simulink model "Template_v5_0_0_2026a_Original"  (R2026a)
settings: Solver=ode4  StopTime=tsim  FixedStep=baseRate  RelTol=1e-6  AbsTol=1e-6
undefined symbols (not defined in the file or in its folder): baseRate, dataRate, DiscIntNeverNeededParam, F_thrusters_BLACK, F_thrusters_BLUE, F_thrusters_RED, home_states_BLACK, home_states_BLUE, home_states_RED, IBLACK, IBLUE, init_states_BLACK, init_states_BLUE, init_states_RED, IRED, K_BLACK, K_BLUE, K_RED, labConsoleIP, mBLACK, mBLUE, mRED, Phase0_End, Phase1_End, Phase2_End, Phase3_End, Phase3_SubPhase1_End, Phase3_SubPhase2_End, Phase3_SubPhase3_End, Phase3_SubPhase4_End, Phase4_End, Phase5_End, platformSelection, PWMFreq, serverRate, simMode, tableDamping_BLACK, tableDamping_BLUE, tableDamping_RED, tableSlope, thrust_decay_BLACK, thrust_decay_BLUE, thrust_decay_RED, thruster_dist2CG_BLACK, thruster_dist2CG_BLUE, thruster_dist2CG_RED, xLength, yLength
libraries: simulink x18, dspinverses x3, nvidiaCommlib x1
(part 5 of 7)

== system Template_v5_0_0_2026a_Original/Simulate Plant Dynamics/BLUE Dynamics/Calculated & Store Measured States/Subsystem1 ==
  dt : Inport
  y : Inport  Port=2
  Constant3 : Constant  Value=0
  Delay1 : Delay  DelayLength=1
  Enabled Subsystem : Subsystem  TreatAsAtomicUnit=on
  Relational Operator : RelationalOperator  Operator=~=  OutDataTypeStr=boolean  RndMeth=Simplest  InputSameDT=off
  Subtract1 : Sum  Inputs=+-
  dy/dt : Outport
  wires:
  Constant3/1 -> Relational Operator/2
  Relational Operator/1 -> Enabled Subsystem/Enable
  Delay1/1 -> Subtract1/2
  dt/1 -> Enabled Subsystem/2(dt)
  Subtract1/1 -> Relational Operator/1
  Enabled Subsystem/1(dy/dt) -> dy/dt/1
  y/1 -> Enabled Subsystem/1(y), Delay1/1, Subtract1/1

== system Template_v5_0_0_2026a_Original/Simulate Plant Dynamics/BLUE Dynamics/Calculated & Store Measured States/Subsystem2 ==
  dt : Inport
  y : Inport  Port=2
  Constant3 : Constant  Value=0
  Delay1 : Delay  DelayLength=1
  Enabled Subsystem : Subsystem  TreatAsAtomicUnit=on
  Relational Operator : RelationalOperator  Operator=~=  OutDataTypeStr=boolean  RndMeth=Simplest  InputSameDT=off
  Subtract1 : Sum  Inputs=+-
  dy/dt : Outport
  wires:
  Constant3/1 -> Relational Operator/2
  Relational Operator/1 -> Enabled Subsystem/Enable
  Delay1/1 -> Subtract1/2
  dt/1 -> Enabled Subsystem/2(dt)
  Subtract1/1 -> Relational Operator/1
  Enabled Subsystem/1(dy/dt) -> dy/dt/1
  y/1 -> Enabled Subsystem/1(y), Delay1/1, Subtract1/1

== system Template_v5_0_0_2026a_Original/Simulate Plant Dynamics/BLUE Dynamics/Calculated & Store Measured States/Wrap ==
  Unwrapped Angle : Inport
  Atan2 : Trigonometry  Operator=atan2
  Cos : Trigonometry  Operator=cos
  Sin : Trigonometry
  Wrapped Angle : Outport
  wires:
  Unwrapped Angle/1 -> Sin/1, Cos/1
  Cos/1 -> Atan2/2
  Atan2/1 -> Wrapped Angle/1
  Sin/1 -> Atan2/1

== system Template_v5_0_0_2026a_Original/Simulate Plant Dynamics/BLUE Dynamics/Calculated & Store True States/Wrap ==
  Unwrapped Angle : Inport
  Atan2 : Trigonometry  Operator=atan2
  Cos : Trigonometry  Operator=cos
  Sin : Trigonometry
  Wrapped Angle : Outport
  wires:
  Unwrapped Angle/1 -> Sin/1, Cos/1
  Cos/1 -> Atan2/2
  Atan2/1 -> Wrapped Angle/1
  Sin/1 -> Atan2/1

== system Template_v5_0_0_2026a_Original/Simulate Plant Dynamics/BLUE Dynamics/Data @ Measurement Rate/Calculate True Time Step ==
  Data : Inport
  Time : Inport  Port=2
  Rate : Inport  Port=3
  Constant3 : Constant  Value=0
  Delay1 : Delay  DelayLength=1  InitialCondition=0
  Delay2 : Delay  DelayLength=1  InitialCondition=0
  Demux : Demux  Outputs=3
  Enabled Subsystem3 : Subsystem  TreatAsAtomicUnit=on
  MATLAB Function : MATLAB Function  TreatAsAtomicUnit=on
  Relational Operator : RelationalOperator  Operator=~=  OutDataTypeStr=boolean  RndMeth=Simplest  InputSameDT=off
  Subtract1 : Sum  Inputs=+-
  Subtract2 : Sum  Inputs=+-
  Terminator : Terminator
  Terminator1 : Terminator
  dt_out : Outport
  wires:
  Demux/3 -> Terminator1/1
  Rate/1 -> MATLAB Function/2(dataRate)
  MATLAB Function/1(dt_out) -> dt_out/1
  Time/1 -> Delay2/1, Subtract1/1
  Enabled Subsystem3/1(dy(t)/dt) -> MATLAB Function/1(dt)
  Data/1 -> Demux/1
  Subtract2/1 -> Relational Operator/1
  Relational Operator/1 -> Enabled Subsystem3/Enable
  Constant3/1 -> Relational Operator/2
  Demux/1 -> Subtract2/1, Delay1/1
  Delay1/1 -> Subtract2/2
  Demux/2 -> Terminator/1
  Subtract1/1 -> Enabled Subsystem3/1(y2-y1)
  Delay2/1 -> Subtract1/2

== system Template_v5_0_0_2026a_Original/Simulate Plant Dynamics/BLUE Dynamics/Data @ Measurement Rate/Enabled Subsystem ==
  In1 : Inport
  Enable : EnablePort
  Out1 : Outport
  wires:
  In1/1 -> Out1/1

== system Template_v5_0_0_2026a_Original/Simulate Plant Dynamics/BLUE Dynamics/Data @ Measurement Rate/Enabled Subsystem1 ==
  ThrustPer_Final : Inport
  Enable : EnablePort
  Out1 : Outport
  wires:
  ThrustPer_Final/1 -> Out1/1

== system Template_v5_0_0_2026a_Original/Simulate Plant Dynamics/RED and ARM Dynamics/RED + ARM/Calculated & Store Measured States ==
  y : Inport
  dt : Inport  Port=2
  Arm (Stored by the Encoder Path) : Terminator
  Demux1 : Demux  Outputs=3
  Demux2 : Demux  Outputs=[3,3]
  Mux3 : Mux  Inputs=3
  Mux4 : Mux  Inputs=3
  Mux5 : Mux  Inputs=2
  Reshape1 : Reshape  OutputDimensionality=Column vector (2-D)
  Subsystem3 : Subsystem
  Subsystem4 : Subsystem
  Subsystem5 : Subsystem
  True States for RED : DataStoreWrite  DataStoreName=RED_Measured_States  IndexOptions=Index vector (dialog)  Indices=1  OutputSizes=1
  Wrap : Subsystem
  wires:
  Demux1/2 -> Mux3/2
  Wrap/1(Wrapped Angle) -> Mux3/3
  Demux2/1 -> Subsystem3/2(y), Demux1/1
  Mux4/1 -> True States for RED/1
  y/1 -> Demux2/1
  Subsystem5/1(dy/dt) -> Mux5/2
  Demux1/1 -> Mux3/1
  Demux2/2 -> Subsystem5/2(y), Mux5/1
  Mux3/1 -> Mux4/1
  Subsystem4/1(dy/dt) -> Mux4/3
  Demux1/3 -> Wrap/1(Unwrapped Angle)
  dt/1 -> Subsystem5/1(dt), Subsystem4/1(dt), Subsystem3/1(dt)
  Reshape1/1 -> Subsystem4/2(y)
  Subsystem3/1(dy/dt) -> Mux4/2, Reshape1/1
  Mux5/1 -> Arm (Stored by the Encoder Path)/1

== system Template_v5_0_0_2026a_Original/Simulate Plant Dynamics/RED and ARM Dynamics/RED + ARM/Calculated & Store True States ==
  y : Inport
  Data Store Write3 : DataStoreWrite  DataStoreName=ARM_True_States  IndexOptions=Index vector (dialog)  Indices=1  OutputSizes=1
  Demux : Demux  Outputs=3
  Demux1 : Demux  Outputs=[3,3]
  Discrete Derivative : simulink/Discrete/Discrete Derivative  gainval=1.0  ICPrevScaledInput=0.0  OutMin=[]  OutMax=[]  OutDataType=fixdt(1, 16)  OutScaling=2^-10  DoSatur=off
  Discrete Derivative1 : simulink/Discrete/Discrete Derivative  gainval=1.0  ICPrevScaledInput=0.0  OutMin=[]  OutMax=[]  OutDataType=fixdt(1, 16)  OutScaling=2^-10  DoSatur=off
  Discrete Derivative2 : simulink/Discrete/Discrete Derivative  gainval=1.0  ICPrevScaledInput=0.0  OutMin=[]  OutMax=[]  OutDataType=fixdt(1, 16)  OutScaling=2^-10  DoSatur=off
  Mux1 : Mux  Inputs=3
  Mux2 : Mux  Inputs=3
  Mux3 : Mux  Inputs=2
  True States for RED : DataStoreWrite  DataStoreName=RED_True_States  IndexOptions=Index vector (dialog)  Indices=1  OutputSizes=1
  Wrap : Subsystem
  wires:
  Demux/1 -> Mux1/1
  Wrap/1(Wrapped Angle) -> Mux1/3
  Demux/3 -> Wrap/1(Unwrapped Angle)
  Demux/2 -> Mux1/2
  Mux2/1 -> True States for RED/1
  Discrete Derivative/1 -> Discrete Derivative1/1, Mux2/2
  Mux1/1 -> Mux2/1
  Discrete Derivative1/1 -> Mux2/3
  y/1 -> Demux1/1
  Demux1/1 -> Discrete Derivative/1, Demux/1
  Mux3/1 -> Data Store Write3/1
  Demux1/2 -> Discrete Derivative2/1, Mux3/1
  Discrete Derivative2/1 -> Mux3/2

== system Template_v5_0_0_2026a_Original/Simulate Plant Dynamics/RED and ARM Dynamics/RED + ARM/Data @ Measurement Rate ==
  Data Input : Inport
  Calculate True Time Step : Subsystem
  Constant1 : Constant  Value=dataRate
  Constant2 : Constant  Value=0
  Data Store Read : DataStoreRead  DataStoreName=Univ_Time  IndexOptions=Index vector (dialog)  Indices=1  OutputSizes=1
  Delay : Delay  DelayLength=1
  Enabled Subsystem : Subsystem  TreatAsAtomicUnit=on
  Enabled Subsystem1 : Subsystem  TreatAsAtomicUnit=on
  Relational Operator1 : RelationalOperator  OutDataTypeStr=boolean  RndMeth=Simplest  InputSameDT=off
  Relational Operator2 : RelationalOperator  Operator===  OutDataTypeStr=boolean  RndMeth=Simplest  InputSameDT=off
  Subtract : Sum  Inputs=+-
  Data Held : Outport
  Time Step : Outport  Port=2
  wires:
  Data Input/1 -> Enabled Subsystem1/1(ThrustPer_Final)
  Subtract/1 -> Relational Operator2/1, Delay/1
  Relational Operator2/1 -> Enabled Subsystem1/Enable
  Relational Operator1/1 -> Enabled Subsystem/Enable
  Constant1/1 -> Calculate True Time Step/3(Rate), Relational Operator1/2
  Constant2/1 -> Relational Operator2/2
  Enabled Subsystem/1(Out1) -> Calculate True Time Step/2(Time), Subtract/2
  Delay/1 -> Relational Operator1/1
  Data Store Read/1 -> Enabled Subsystem/1(In1), Subtract/1
  Enabled Subsystem1/1(Out1) -> Calculate True Time Step/1(Data), Data Held/1
  Calculate True Time Step/1(dt_out) -> Time Step/1

== system Template_v5_0_0_2026a_Original/Simulate Plant Dynamics/RED and ARM Dynamics/RED + ARM/Exceeded Table Limits ==
  X : Inport
  Y : Inport  Port=2
  Constant : Constant  Value=xLength
  Constant1 : Constant  Value=0
  Constant2 : Constant  Value=yLength
  Constant3 : Constant  Value=0
  Logical Operator : Logic  Operator=OR  AllPortsSameDT=off  OutDataTypeStr=boolean
  Logical Operator1 : Logic  Operator=OR  AllPortsSameDT=off  OutDataTypeStr=boolean
  Logical Operator2 : Logic  Operator=OR  AllPortsSameDT=off  OutDataTypeStr=boolean
  Relational Operator : RelationalOperator  OutDataTypeStr=boolean  RndMeth=Simplest  InputSameDT=off
  Relational Operator1 : RelationalOperator  Operator=<  OutDataTypeStr=boolean  RndMeth=Simplest  InputSameDT=off
  Relational Operator2 : RelationalOperator  OutDataTypeStr=boolean  RndMeth=Simplest  InputSameDT=off
  Relational Operator3 : RelationalOperator  Operator=<  OutDataTypeStr=boolean  RndMeth=Simplest  InputSameDT=off
  Stop : Outport
  wires:
  Constant1/1 -> Relational Operator1/2
  Relational Operator/1 -> Logical Operator/1
  Relational Operator1/1 -> Logical Operator/2
  Constant/1 -> Relational Operator/2
  X/1 -> Relational Operator1/1, Relational Operator/1
  Relational Operator3/1 -> Logical Operator1/2
  Relational Operator2/1 -> Logical Operator1/1
  Constant3/1 -> Relational Operator3/2
  Constant2/1 -> Relational Operator2/2
  Y/1 -> Relational Operator3/1, Relational Operator2/1
  Logical Operator2/1 -> Stop/1
  Logical Operator/1 -> Logical Operator2/1
  Logical Operator1/1 -> Logical Operator2/2

== system Template_v5_0_0_2026a_Original/Simulate Plant Dynamics/RED and ARM Dynamics/RED Only/Calculated & Store Measured States ==
  y : Inport
  dt : Inport  Port=2
  Demux : Demux  Outputs=3
  Measured States for RED : DataStoreWrite  DataStoreName=RED_Measured_States  IndexOptions=Index vector (dialog)  Indices=1  OutputSizes=1
  Mux1 : Mux  Inputs=3
  Mux2 : Mux  Inputs=3
  Reshape : Reshape  OutputDimensionality=Column vector (2-D)
  Subsystem1 : Subsystem
  Subsystem2 : Subsystem
  Wrap : Subsystem
  wires:
  Demux/1 -> Mux1/1
  Wrap/1(Wrapped Angle) -> Mux1/3
  Demux/3 -> Wrap/1(Unwrapped Angle)
  Demux/2 -> Mux1/2
  Reshape/1 -> Subsystem1/2(y)
  dt/1 -> Subsystem2/1(dt), Subsystem1/1(dt)
  y/1 -> Subsystem2/2(y), Demux/1
  Mux1/1 -> Mux2/1
  Subsystem1/1(dy/dt) -> Mux2/3
  Mux2/1 -> Measured States for RED/1
  Subsystem2/1(dy/dt) -> Mux2/2, Reshape/1

== system Template_v5_0_0_2026a_Original/Simulate Plant Dynamics/RED and ARM Dynamics/RED Only/Calculated & Store True States ==
  y : Inport
  Demux : Demux  Outputs=3
  Discrete Derivative : simulink/Discrete/Discrete Derivative  gainval=1.0  ICPrevScaledInput=0.0  OutMin=[]  OutMax=[]  OutDataType=fixdt(1, 16)  OutScaling=2^-10  DoSatur=off
  Discrete Derivative1 : simulink/Discrete/Discrete Derivative  gainval=1.0  ICPrevScaledInput=0.0  OutMin=[]  OutMax=[]  OutDataType=fixdt(1, 16)  OutScaling=2^-10  DoSatur=off
  Mux1 : Mux  Inputs=3
  Mux2 : Mux  Inputs=3
  True States for RED : DataStoreWrite  DataStoreName=RED_True_States  IndexOptions=Index vector (dialog)  Indices=1  OutputSizes=1
  Wrap : Subsystem
  wires:
  Demux/1 -> Mux1/1
  Wrap/1(Wrapped Angle) -> Mux1/3
  Demux/3 -> Wrap/1(Unwrapped Angle)
  Demux/2 -> Mux1/2
  Mux2/1 -> True States for RED/1
  y/1 -> Discrete Derivative/1, Demux/1
  Discrete Derivative/1 -> Mux2/2, Discrete Derivative1/1
  Mux1/1 -> Mux2/1
  Discrete Derivative1/1 -> Mux2/3

== system Template_v5_0_0_2026a_Original/Simulate Plant Dynamics/RED and ARM Dynamics/RED Only/Data @ Measurement Rate ==
  Data Input : Inport
  Calculate True Time Step : Subsystem
  Constant1 : Constant  Value=dataRate
  Constant2 : Constant  Value=0
  Data Store Read : DataStoreRead  DataStoreName=Univ_Time  IndexOptions=Index vector (dialog)  Indices=1  OutputSizes=1
  Delay : Delay  DelayLength=1
  Enabled Subsystem : Subsystem  TreatAsAtomicUnit=on
  Enabled Subsystem1 : Subsystem  TreatAsAtomicUnit=on
  Relational Operator1 : RelationalOperator  OutDataTypeStr=boolean  RndMeth=Simplest  InputSameDT=off
  Relational Operator2 : RelationalOperator  Operator===  OutDataTypeStr=boolean  RndMeth=Simplest  InputSameDT=off
  Subtract : Sum  Inputs=+-
  Data Held : Outport
  Time Step : Outport  Port=2
  wires:
  Data Input/1 -> Enabled Subsystem1/1(ThrustPer_Final)
  Subtract/1 -> Relational Operator2/1, Delay/1
  Relational Operator2/1 -> Enabled Subsystem1/Enable
  Relational Operator1/1 -> Enabled Subsystem/Enable
  Constant1/1 -> Calculate True Time Step/3(Rate), Relational Operator1/2
  Constant2/1 -> Relational Operator2/2
  Enabled Subsystem/1(Out1) -> Calculate True Time Step/2(Time), Subtract/2
  Delay/1 -> Relational Operator1/1
  Data Store Read/1 -> Enabled Subsystem/1(In1), Subtract/1
  Enabled Subsystem1/1(Out1) -> Calculate True Time Step/1(Data), Data Held/1
  Calculate True Time Step/1(dt_out) -> Time Step/1

== system Template_v5_0_0_2026a_Original/Simulate Plant Dynamics/RED and ARM Dynamics/RED Only/Dynamics Model for RED ==
  control_inputs : Inport
  Acceleration to Velocity : DiscreteIntegrator  IntegratorMethod=Integration: Backward Euler  SampleTime=-1  ICPrevOutput=DiscIntNeverNeededParam  ICPrevScaledInput=DiscIntNeverNeededParam
  Float State : DataStoreRead  DataStoreName=Float_State  IndexOptions=Index vector (dialog)  Indices=1  OutputSizes=1
  MATLAB Function : MATLAB Function  TreatAsAtomicUnit=on
  Previous Position : UnitDelay  InitialCondition=init_states_RED(:)  SampleTime=-1
  Previous Velocity : UnitDelay  InitialCondition=[0; 0; 0]  SampleTime=-1
  Velocity to Position : DiscreteIntegrator  IntegratorMethod=Integration: Backward Euler  InitialCondition=init_states_RED  SampleTime=-1  ICPrevOutput=DiscIntNeverNeededParam  ICPrevScaledInput=DiscIntNeverNeededParam
  states : Outport  VectorParamsAs1DForOutWhenUnconnected=off
  wires:
  control_inputs/1 -> MATLAB Function/1(control_inputs)
  MATLAB Function/1(x_ddot) -> Acceleration to Velocity/1
  Acceleration to Velocity/1 -> Velocity to Position/1, Previous Velocity/1
  Velocity to Position/1 -> states/1, Previous Position/1
  Previous Position/1 -> MATLAB Function/2(position)
  Previous Velocity/1 -> MATLAB Function/3(velocity)
  Float State/1 -> MATLAB Function/4(floating)

== system Template_v5_0_0_2026a_Original/Thruster & Float Control Code/Change BLACK Behavior/Calculate Duty Cycle/Duty Cycle @ PWM ==
  ThrustPer_Final : Inport
  Constant1 : Constant  Value=1/PWMFreq
  Constant2 : Constant  Value=0
  Data Store Read : DataStoreRead  DataStoreName=Univ_Time  IndexOptions=Index vector (dialog)  Indices=1  OutputSizes=1
  Delay : Delay  DelayLength=1
  Enabled Subsystem : Subsystem  TreatAsAtomicUnit=on
  Enabled Subsystem1 : Subsystem  TreatAsAtomicUnit=on
  Relational Operator1 : RelationalOperator  OutDataTypeStr=boolean  RndMeth=Simplest  InputSameDT=off
  Relational Operator2 : RelationalOperator  Operator===  OutDataTypeStr=boolean  RndMeth=Simplest  InputSameDT=off
  Subtract : Sum  Inputs=+-
  Duty Cycle Held : Outport
  wires:
  Data Store Read/1 -> Enabled Subsystem/1(In1), Subtract/1
  ThrustPer_Final/1 -> Enabled Subsystem1/1(ThrustPer_Final)
  Subtract/1 -> Relational Operator2/1, Delay/1
  Relational Operator2/1 -> Enabled Subsystem1/Enable
  Relational Operator1/1 -> Enabled Subsystem/Enable
  Constant1/1 -> Relational Operator1/2
  Constant2/1 -> Relational Operator2/2
  Enabled Subsystem/1(Out1) -> Subtract/2
  Enabled Subsystem1/1(Out1) -> Duty Cycle Held/1
  Delay/1 -> Relational Operator1/1

== system Template_v5_0_0_2026a_Original/Thruster & Float Control Code/Change BLACK Behavior/Calculate Duty Cycle/Generate Initial Guess ==
  "[Fx; Fy; Tz]" : Inport
  MATLAB Function : MATLAB Function  TreatAsAtomicUnit=on
  Product3 : Product  Multiplication=Matrix(*)
  Pseudoinverse1 : dspinverses/Pseudoinverse  wanterr=off  SimulateUsing=Interpreted execution
  Duty Cycle : Outport
  wires:
  Pseudoinverse1/1 -> Product3/1
  MATLAB Function/1(H) -> Pseudoinverse1/1
  Product3/1 -> Duty Cycle/1
  "[Fx; Fy; Tz]"/1 -> Product3/2

== system Template_v5_0_0_2026a_Original/Thruster & Float Control Code/Change BLACK Behavior/Calculate Duty Cycle/Rotate Forces to Inertial ==
  "F_b " : Inport
  Rz : Inport  Port=2
  Create Rotation Matrix : MATLAB Function  TreatAsAtomicUnit=on
  Rotate F_b to F_I : Product  Multiplication=Matrix(*)
  F_I : Outport  VectorParamsAs1DForOutWhenUnconnected=off
  wires:
  "F_b "/1 -> Rotate F_b to F_I/2
  Rotate F_b to F_I/1 -> F_I/1
  Create Rotation Matrix/1(C_Ib) -> Rotate F_b to F_I/1
  Rz/1 -> Create Rotation Matrix/1(Rz)

== system Template_v5_0_0_2026a_Original/Thruster & Float Control Code/Change BLUE Behavior/Calculate Duty Cycle/Duty Cycle @ PWM ==
  ThrustPer_Final : Inport
  Constant1 : Constant  Value=1/PWMFreq
  Constant2 : Constant  Value=0
  Data Store Read : DataStoreRead  DataStoreName=Univ_Time  IndexOptions=Index vector (dialog)  Indices=1  OutputSizes=1
  Delay : Delay  DelayLength=1
  Enabled Subsystem : Subsystem  TreatAsAtomicUnit=on
  Enabled Subsystem1 : Subsystem  TreatAsAtomicUnit=on
  Relational Operator1 : RelationalOperator  OutDataTypeStr=boolean  RndMeth=Simplest  InputSameDT=off
  Relational Operator2 : RelationalOperator  Operator===  OutDataTypeStr=boolean  RndMeth=Simplest  InputSameDT=off
  Subtract : Sum  Inputs=+-
  Duty Cycle Held : Outport
  wires:
  Data Store Read/1 -> Enabled Subsystem/1(In1), Subtract/1
  ThrustPer_Final/1 -> Enabled Subsystem1/1(ThrustPer_Final)
  Subtract/1 -> Relational Operator2/1, Delay/1
  Relational Operator2/1 -> Enabled Subsystem1/Enable
  Relational Operator1/1 -> Enabled Subsystem/Enable
  Constant1/1 -> Relational Operator1/2
  Constant2/1 -> Relational Operator2/2
  Enabled Subsystem/1(Out1) -> Subtract/2
  Enabled Subsystem1/1(Out1) -> Duty Cycle Held/1
  Delay/1 -> Relational Operator1/1

== system Template_v5_0_0_2026a_Original/Thruster & Float Control Code/Change BLUE Behavior/Calculate Duty Cycle/Generate Initial Guess ==
  "[Fx; Fy; Tz]" : Inport
  MATLAB Function : MATLAB Function  TreatAsAtomicUnit=on
  Product3 : Product  Multiplication=Matrix(*)
  Pseudoinverse1 : dspinverses/Pseudoinverse  wanterr=off  SimulateUsing=Interpreted execution
  Duty Cycle : Outport
  wires:
  Pseudoinverse1/1 -> Product3/1
  MATLAB Function/1(H) -> Pseudoinverse1/1
  Product3/1 -> Duty Cycle/1
  "[Fx; Fy; Tz]"/1 -> Product3/2

== system Template_v5_0_0_2026a_Original/Thruster & Float Control Code/Change BLUE Behavior/Calculate Duty Cycle/Rotate Forces to Inertial ==
  "F_b " : Inport
  Rz : Inport  Port=2
  Create Rotation Matrix : MATLAB Function  TreatAsAtomicUnit=on
  Rotate F_b to F_I : Product  Multiplication=Matrix(*)
  F_I : Outport  VectorParamsAs1DForOutWhenUnconnected=off
  wires:
  "F_b "/1 -> Rotate F_b to F_I/2
  Rotate F_b to F_I/1 -> F_I/1
  Create Rotation Matrix/1(C_Ib) -> Rotate F_b to F_I/1
  Rz/1 -> Create Rotation Matrix/1(Rz)

== system Template_v5_0_0_2026a_Original/Thruster & Float Control Code/Change RED Behavior/Calculate Duty Cycle/Duty Cycle @ PWM ==
  ThrustPer_Final : Inport
  Constant1 : Constant  Value=1/PWMFreq
  Constant2 : Constant  Value=0
  Data Store Read : DataStoreRead  DataStoreName=Univ_Time  IndexOptions=Index vector (dialog)  Indices=1  OutputSizes=1
  Delay : Delay  DelayLength=1
  Enabled Subsystem : Subsystem  TreatAsAtomicUnit=on
  Enabled Subsystem1 : Subsystem  TreatAsAtomicUnit=on
  Relational Operator1 : RelationalOperator  OutDataTypeStr=boolean  RndMeth=Simplest  InputSameDT=off
  Relational Operator2 : RelationalOperator  Operator===  OutDataTypeStr=boolean  RndMeth=Simplest  InputSameDT=off
  Subtract : Sum  Inputs=+-
  Duty Cycle Held : Outport
  wires:
  Data Store Read/1 -> Enabled Subsystem/1(In1), Subtract/1
  ThrustPer_Final/1 -> Enabled Subsystem1/1(ThrustPer_Final)
  Subtract/1 -> Relational Operator2/1, Delay/1
  Relational Operator2/1 -> Enabled Subsystem1/Enable
  Relational Operator1/1 -> Enabled Subsystem/Enable
  Constant1/1 -> Relational Operator1/2
  Constant2/1 -> Relational Operator2/2
  Enabled Subsystem/1(Out1) -> Subtract/2
  Enabled Subsystem1/1(Out1) -> Duty Cycle Held/1
  Delay/1 -> Relational Operator1/1

== system Template_v5_0_0_2026a_Original/Thruster & Float Control Code/Change RED Behavior/Calculate Duty Cycle/Generate Initial Guess ==
  "[Fx; Fy; Tz]" : Inport
  MATLAB Function : MATLAB Function  TreatAsAtomicUnit=on
  Product3 : Product  Multiplication=Matrix(*)
  Pseudoinverse1 : dspinverses/Pseudoinverse  wanterr=off  SimulateUsing=Interpreted execution
  Duty Cycle : Outport
  wires:
  Pseudoinverse1/1 -> Product3/1
  MATLAB Function/1(H) -> Pseudoinverse1/1
  Product3/1 -> Duty Cycle/1
  "[Fx; Fy; Tz]"/1 -> Product3/2

== system Template_v5_0_0_2026a_Original/Thruster & Float Control Code/Change RED Behavior/Calculate Duty Cycle/Rotate Forces to Inertial ==
  "F_b " : Inport
  Rz : Inport  Port=2
  Create Rotation Matrix : MATLAB Function  TreatAsAtomicUnit=on
  Rotate F_b to F_I : Product  Multiplication=Matrix(*)
  F_I : Outport  VectorParamsAs1DForOutWhenUnconnected=off
  wires:
  "F_b "/1 -> Rotate F_b to F_I/2
  Rotate F_b to F_I/1 -> F_I/1
  Create Rotation Matrix/1(C_Ib) -> Rotate F_b to F_I/1
  Rz/1 -> Create Rotation Matrix/1(Rz)

== system Template_v5_0_0_2026a_Original/1 - Experiment Logic/Phase #3: Experiment/Sub-Phase #1/Desired Position BLACK/Calculate Circular Tracking ==
  Angular Frequency : Inport
  Phase : Inport  Port=2
  Constant1 : Constant  Value=xLength/2
  Constant2 : Constant  Value=yLength/2
  Cos : Trigonometry  Operator=cos
  Gain : Gain  Gain=0.85
  Gain1 : Gain  Gain=0.85
  Sin : Trigonometry
  Sum{,1..3} (4 alike) : Sum  Inputs=|++
  Target X : Outport
  Target Y : Outport  Port=2
  wires:
  Constant2/1 -> Sum2/2
  Constant1/1 -> Sum1/2
  Cos/1 -> Gain/1
  Gain1/1 -> Sum2/1
  Sin/1 -> Gain1/1
  Gain/1 -> Sum1/1
  Sum2/1 -> Target Y/1
  Sum1/1 -> Target X/1
  Angular Frequency/1 -> Sum3/1, Sum/1
  Sum/1 -> Cos/1
  Phase/1 -> Sum3/2, Sum/2
  Sum3/1 -> Sin/1

== system Template_v5_0_0_2026a_Original/1 - Experiment Logic/Phase #3: Experiment/Sub-Phase #1/Desired Position BLACK/Calculate Time since Phase #3 Start ==
  Constant2 : Constant  Value=Phase2_End  SampleTime=-1
  Subsystem : Subsystem
  Subtract3 : Sum  Inputs=+-
  Time : Outport  VectorParamsAs1DForOutWhenUnconnected=off
  wires:
  Subtract3/1 -> Time/1
  Constant2/1 -> Subtract3/2
  Subsystem/1(Time) -> Subtract3/1

== system Template_v5_0_0_2026a_Original/1 - Experiment Logic/Phase #3: Experiment/Sub-Phase #1/Desired Position BLACK/Wrap ==
  In1 : Inport
  Atan2 : Trigonometry  Operator=atan2
  Cos : Trigonometry  Operator=cos
  Sin : Trigonometry
  Out1 : Outport
  wires:
  In1/1 -> Sin/1, Cos/1
  Cos/1 -> Atan2/2
  Atan2/1 -> Out1/1
  Sin/1 -> Atan2/1

== system Template_v5_0_0_2026a_Original/1 - Experiment Logic/Phase #3: Experiment/Sub-Phase #1/Desired Position BLUE/Calculate Circular Tracking ==
  Angular Frequency : Inport
  Phase : Inport  Port=2
  Constant1 : Constant  Value=xLength/2
  Constant2 : Constant  Value=yLength/2
  Cos : Trigonometry  Operator=cos
  Gain : Gain  Gain=0.85
  Gain1 : Gain  Gain=0.85
  Sin : Trigonometry
  Sum{,1..3} (4 alike) : Sum  Inputs=|++
  Target X : Outport
  Target Y : Outport  Port=2
  wires:
  Constant2/1 -> Sum2/2
  Constant1/1 -> Sum1/2
  Cos/1 -> Gain/1
  Gain1/1 -> Sum2/1
  Sin/1 -> Gain1/1
  Gain/1 -> Sum1/1
  Sum2/1 -> Target Y/1
  Sum1/1 -> Target X/1
  Angular Frequency/1 -> Sum3/1, Sum/1
  Sum/1 -> Cos/1
  Phase/1 -> Sum3/2, Sum/2
  Sum3/1 -> Sin/1

== system Template_v5_0_0_2026a_Original/1 - Experiment Logic/Phase #3: Experiment/Sub-Phase #1/Desired Position BLUE/Calculate Time since Phase #3 Start ==
  Constant2 : Constant  Value=Phase2_End  SampleTime=-1
  Subsystem : Subsystem
  Subtract3 : Sum  Inputs=+-
  Time : Outport  VectorParamsAs1DForOutWhenUnconnected=off
  wires:
  Subtract3/1 -> Time/1
  Constant2/1 -> Subtract3/2
  Subsystem/1(Time) -> Subtract3/1

== system Template_v5_0_0_2026a_Original/1 - Experiment Logic/Phase #3: Experiment/Sub-Phase #1/Desired Position BLUE/Wrap ==
  In1 : Inport
  Atan2 : Trigonometry  Operator=atan2
  Cos : Trigonometry  Operator=cos
  Sin : Trigonometry
  Out1 : Outport
  wires:
  In1/1 -> Sin/1, Cos/1
  Cos/1 -> Atan2/2
  Atan2/1 -> Out1/1
  Sin/1 -> Atan2/1

== system Template_v5_0_0_2026a_Original/1 - Experiment Logic/Phase #3: Experiment/Sub-Phase #1/Desired Position RED/Calculate Circular Tracking ==
  Angular Frequency : Inport
  Phase : Inport  Port=2
  Constant1 : Constant  Value=xLength/2
  Constant2 : Constant  Value=yLength/2
  Cos : Trigonometry  Operator=cos
  Gain : Gain  Gain=0.85
  Gain1 : Gain  Gain=0.85
  Sin : Trigonometry
  Sum{,1..3} (4 alike) : Sum  Inputs=|++
  Target X : Outport
  Target Y : Outport  Port=2
  wires:
  Constant2/1 -> Sum2/2
  Constant1/1 -> Sum1/2
  Cos/1 -> Gain/1
  Gain1/1 -> Sum2/1
  Sin/1 -> Gain1/1
  Gain/1 -> Sum1/1
  Sum2/1 -> Target Y/1
  Sum1/1 -> Target X/1
  Angular Frequency/1 -> Sum3/1, Sum/1
  Sum/1 -> Cos/1
  Phase/1 -> Sum3/2, Sum/2
  Sum3/1 -> Sin/1

== system Template_v5_0_0_2026a_Original/1 - Experiment Logic/Phase #3: Experiment/Sub-Phase #1/Desired Position RED/Calculate Time since Phase #3 Start ==
  Constant2 : Constant  Value=Phase2_End  SampleTime=-1
  Subsystem : Subsystem
  Subtract3 : Sum  Inputs=+-
  Time : Outport  VectorParamsAs1DForOutWhenUnconnected=off
  wires:
  Subtract3/1 -> Time/1
  Constant2/1 -> Subtract3/2
  Subsystem/1(Time) -> Subtract3/1

== system Template_v5_0_0_2026a_Original/1 - Experiment Logic/Phase #3: Experiment/Sub-Phase #1/Desired Position RED/Wrap ==
  In1 : Inport
  Atan2 : Trigonometry  Operator=atan2
  Cos : Trigonometry  Operator=cos
  Sin : Trigonometry
  Out1 : Outport
  wires:
  In1/1 -> Sin/1, Cos/1
  Cos/1 -> Atan2/2
  Atan2/1 -> Out1/1
  Sin/1 -> Atan2/1

== system Template_v5_0_0_2026a_Original/1 - Experiment Logic/Phase #3: Experiment/Sub-Phase #2/Desired Position BLACK/Calculate Circular Tracking ==
  Angular Frequency : Inport
  Phase : Inport  Port=2
  Constant1 : Constant  Value=xLength/2
  Constant2 : Constant  Value=yLength/2
  Cos : Trigonometry  Operator=cos
  Gain : Gain  Gain=0.85
  Gain1 : Gain  Gain=0.85
  Sin : Trigonometry
  Sum{,1..3} (4 alike) : Sum  Inputs=|++
  Target X : Outport
  Target Y : Outport  Port=2
  wires:
  Constant2/1 -> Sum2/2
  Constant1/1 -> Sum1/2
  Cos/1 -> Gain/1
  Gain1/1 -> Sum2/1
  Sin/1 -> Gain1/1
  Gain/1 -> Sum1/1
  Sum2/1 -> Target Y/1
  Sum1/1 -> Target X/1
  Angular Frequency/1 -> Sum3/1, Sum/1
  Sum/1 -> Cos/1
  Phase/1 -> Sum3/2, Sum/2
  Sum3/1 -> Sin/1

== system Template_v5_0_0_2026a_Original/1 - Experiment Logic/Phase #3: Experiment/Sub-Phase #2/Desired Position BLACK/Calculate Time since Phase #3 Start ==
  Constant2 : Constant  Value=Phase2_End  SampleTime=-1
  Subsystem : Subsystem
  Subtract3 : Sum  Inputs=+-
  Time : Outport  VectorParamsAs1DForOutWhenUnconnected=off
  wires:
  Subtract3/1 -> Time/1
  Constant2/1 -> Subtract3/2
  Subsystem/1(Time) -> Subtract3/1

== system Template_v5_0_0_2026a_Original/1 - Experiment Logic/Phase #3: Experiment/Sub-Phase #2/Desired Position BLACK/Wrap ==
  In1 : Inport
  Atan2 : Trigonometry  Operator=atan2
  Cos : Trigonometry  Operator=cos
  Sin : Trigonometry
  Out1 : Outport
  wires:
  In1/1 -> Sin/1, Cos/1
  Cos/1 -> Atan2/2
  Atan2/1 -> Out1/1
  Sin/1 -> Atan2/1

== system Template_v5_0_0_2026a_Original/1 - Experiment Logic/Phase #3: Experiment/Sub-Phase #2/Desired Position BLUE/Calculate Circular Tracking ==
  Angular Frequency : Inport
  Phase : Inport  Port=2
  Constant1 : Constant  Value=xLength/2
  Constant2 : Constant  Value=yLength/2
  Cos : Trigonometry  Operator=cos
  Gain : Gain  Gain=0.85
  Gain1 : Gain  Gain=0.85
  Sin : Trigonometry
  Sum{,1..3} (4 alike) : Sum  Inputs=|++
  Target X : Outport
  Target Y : Outport  Port=2
  wires:
  Constant2/1 -> Sum2/2
  Constant1/1 -> Sum1/2
  Cos/1 -> Gain/1
  Gain1/1 -> Sum2/1
  Sin/1 -> Gain1/1
  Gain/1 -> Sum1/1
  Sum2/1 -> Target Y/1
  Sum1/1 -> Target X/1
  Angular Frequency/1 -> Sum3/1, Sum/1
  Sum/1 -> Cos/1
  Phase/1 -> Sum3/2, Sum/2
  Sum3/1 -> Sin/1

== system Template_v5_0_0_2026a_Original/1 - Experiment Logic/Phase #3: Experiment/Sub-Phase #2/Desired Position BLUE/Calculate Time since Phase #3 Start ==
  Constant2 : Constant  Value=Phase2_End  SampleTime=-1
  Subsystem : Subsystem
  Subtract3 : Sum  Inputs=+-
  Time : Outport  VectorParamsAs1DForOutWhenUnconnected=off
  wires:
  Subtract3/1 -> Time/1
  Constant2/1 -> Subtract3/2
  Subsystem/1(Time) -> Subtract3/1

== system Template_v5_0_0_2026a_Original/1 - Experiment Logic/Phase #3: Experiment/Sub-Phase #2/Desired Position BLUE/Wrap ==
  In1 : Inport
  Atan2 : Trigonometry  Operator=atan2
  Cos : Trigonometry  Operator=cos
  Sin : Trigonometry
  Out1 : Outport
  wires:
  In1/1 -> Sin/1, Cos/1
  Cos/1 -> Atan2/2
  Atan2/1 -> Out1/1
  Sin/1 -> Atan2/1

== system Template_v5_0_0_2026a_Original/1 - Experiment Logic/Phase #3: Experiment/Sub-Phase #2/Desired Position RED/Calculate Circular Tracking ==
  Angular Frequency : Inport
  Phase : Inport  Port=2
  Constant1 : Constant  Value=xLength/2
  Constant2 : Constant  Value=yLength/2
  Cos : Trigonometry  Operator=cos
  Gain : Gain  Gain=0.85
  Gain1 : Gain  Gain=0.85
  Sin : Trigonometry
  Sum{,1..3} (4 alike) : Sum  Inputs=|++
  Target X : Outport
  Target Y : Outport  Port=2
  wires:
  Constant2/1 -> Sum2/2
  Constant1/1 -> Sum1/2
  Cos/1 -> Gain/1
  Gain1/1 -> Sum2/1
  Sin/1 -> Gain1/1
  Gain/1 -> Sum1/1
  Sum2/1 -> Target Y/1
  Sum1/1 -> Target X/1
  Angular Frequency/1 -> Sum3/1, Sum/1
  Sum/1 -> Cos/1
  Phase/1 -> Sum3/2, Sum/2
  Sum3/1 -> Sin/1

== system Template_v5_0_0_2026a_Original/1 - Experiment Logic/Phase #3: Experiment/Sub-Phase #2/Desired Position RED/Calculate Time since Phase #3 Start ==
  Constant2 : Constant  Value=Phase2_End  SampleTime=-1
  Subsystem : Subsystem
  Subtract3 : Sum  Inputs=+-
  Time : Outport  VectorParamsAs1DForOutWhenUnconnected=off
  wires:
  Subtract3/1 -> Time/1
  Constant2/1 -> Subtract3/2
  Subsystem/1(Time) -> Subtract3/1

== system Template_v5_0_0_2026a_Original/1 - Experiment Logic/Phase #3: Experiment/Sub-Phase #2/Desired Position RED/Wrap ==
  In1 : Inport
  Atan2 : Trigonometry  Operator=atan2
  Cos : Trigonometry  Operator=cos
  Sin : Trigonometry
  Out1 : Outport
  wires:
  In1/1 -> Sin/1, Cos/1
  Cos/1 -> Atan2/2
  Atan2/1 -> Out1/1
  Sin/1 -> Atan2/1

== system Template_v5_0_0_2026a_Original/1 - Experiment Logic/Phase #3: Experiment/Sub-Phase #3/Desired Position BLACK/Calculate Circular Tracking ==
  Angular Frequency : Inport
  Phase : Inport  Port=2
  Constant1 : Constant  Value=xLength/2
  Constant2 : Constant  Value=yLength/2
  Cos : Trigonometry  Operator=cos
  Gain : Gain  Gain=0.85
  Gain1 : Gain  Gain=0.85
  Sin : Trigonometry
  Sum{,1..3} (4 alike) : Sum  Inputs=|++
  Target X : Outport
  Target Y : Outport  Port=2
  wires:
  Constant2/1 -> Sum2/2
  Constant1/1 -> Sum1/2
  Cos/1 -> Gain/1
  Gain1/1 -> Sum2/1
  Sin/1 -> Gain1/1
  Gain/1 -> Sum1/1
  Sum2/1 -> Target Y/1
  Sum1/1 -> Target X/1
  Angular Frequency/1 -> Sum3/1, Sum/1
  Sum/1 -> Cos/1
  Phase/1 -> Sum3/2, Sum/2
  Sum3/1 -> Sin/1

== system Template_v5_0_0_2026a_Original/1 - Experiment Logic/Phase #3: Experiment/Sub-Phase #3/Desired Position BLACK/Calculate Time since Phase #3 Start ==
  Constant2 : Constant  Value=Phase2_End  SampleTime=-1
  Subsystem : Subsystem
  Subtract3 : Sum  Inputs=+-
  Time : Outport  VectorParamsAs1DForOutWhenUnconnected=off
  wires:
  Subtract3/1 -> Time/1
  Constant2/1 -> Subtract3/2
  Subsystem/1(Time) -> Subtract3/1

== system Template_v5_0_0_2026a_Original/1 - Experiment Logic/Phase #3: Experiment/Sub-Phase #3/Desired Position BLACK/Wrap ==
  In1 : Inport
  Atan2 : Trigonometry  Operator=atan2
  Cos : Trigonometry  Operator=cos
  Sin : Trigonometry
  Out1 : Outport
  wires:
  In1/1 -> Sin/1, Cos/1
  Cos/1 -> Atan2/2
  Atan2/1 -> Out1/1
  Sin/1 -> Atan2/1

== system Template_v5_0_0_2026a_Original/1 - Experiment Logic/Phase #3: Experiment/Sub-Phase #3/Desired Position BLUE/Calculate Circular Tracking ==
  Angular Frequency : Inport
  Phase : Inport  Port=2
  Constant1 : Constant  Value=xLength/2
  Constant2 : Constant  Value=yLength/2
  Cos : Trigonometry  Operator=cos
  Gain : Gain  Gain=0.85
  Gain1 : Gain  Gain=0.85
  Sin : Trigonometry
  Sum{,1..3} (4 alike) : Sum  Inputs=|++
  Target X : Outport
  Target Y : Outport  Port=2
  wires:
  Constant2/1 -> Sum2/2
  Constant1/1 -> Sum1/2
  Cos/1 -> Gain/1
  Gain1/1 -> Sum2/1
  Sin/1 -> Gain1/1
  Gain/1 -> Sum1/1
  Sum2/1 -> Target Y/1
  Sum1/1 -> Target X/1
  Angular Frequency/1 -> Sum3/1, Sum/1
  Sum/1 -> Cos/1
  Phase/1 -> Sum3/2, Sum/2
  Sum3/1 -> Sin/1

== system Template_v5_0_0_2026a_Original/1 - Experiment Logic/Phase #3: Experiment/Sub-Phase #3/Desired Position BLUE/Calculate Time since Phase #3 Start ==
  Constant2 : Constant  Value=Phase2_End  SampleTime=-1
  Subsystem : Subsystem
  Subtract3 : Sum  Inputs=+-
  Time : Outport  VectorParamsAs1DForOutWhenUnconnected=off
  wires:
  Subtract3/1 -> Time/1
  Constant2/1 -> Subtract3/2
  Subsystem/1(Time) -> Subtract3/1

== system Template_v5_0_0_2026a_Original/1 - Experiment Logic/Phase #3: Experiment/Sub-Phase #3/Desired Position BLUE/Wrap ==
  In1 : Inport
  Atan2 : Trigonometry  Operator=atan2
  Cos : Trigonometry  Operator=cos
  Sin : Trigonometry
  Out1 : Outport
  wires:
  In1/1 -> Sin/1, Cos/1
  Cos/1 -> Atan2/2
  Atan2/1 -> Out1/1
  Sin/1 -> Atan2/1

== system Template_v5_0_0_2026a_Original/1 - Experiment Logic/Phase #3: Experiment/Sub-Phase #3/Desired Position RED/Calculate Circular Tracking ==
  Angular Frequency : Inport
  Phase : Inport  Port=2
  Constant1 : Constant  Value=xLength/2
  Constant2 : Constant  Value=yLength/2
  Cos : Trigonometry  Operator=cos
  Gain : Gain  Gain=0.85
  Gain1 : Gain  Gain=0.85
  Sin : Trigonometry
  Sum{,1..3} (4 alike) : Sum  Inputs=|++
  Target X : Outport
  Target Y : Outport  Port=2
  wires:
  Constant2/1 -> Sum2/2
  Constant1/1 -> Sum1/2
  Cos/1 -> Gain/1
  Gain1/1 -> Sum2/1
  Sin/1 -> Gain1/1
  Gain/1 -> Sum1/1
  Sum2/1 -> Target Y/1
  Sum1/1 -> Target X/1
  Angular Frequency/1 -> Sum3/1, Sum/1
  Sum/1 -> Cos/1
  Phase/1 -> Sum3/2, Sum/2
  Sum3/1 -> Sin/1

== system Template_v5_0_0_2026a_Original/1 - Experiment Logic/Phase #3: Experiment/Sub-Phase #3/Desired Position RED/Calculate Time since Phase #3 Start ==
  Constant2 : Constant  Value=Phase2_End  SampleTime=-1
  Subsystem : Subsystem
  Subtract3 : Sum  Inputs=+-
  Time : Outport  VectorParamsAs1DForOutWhenUnconnected=off
  wires:
  Subtract3/1 -> Time/1
  Constant2/1 -> Subtract3/2
  Subsystem/1(Time) -> Subtract3/1

== system Template_v5_0_0_2026a_Original/1 - Experiment Logic/Phase #3: Experiment/Sub-Phase #3/Desired Position RED/Wrap ==
  In1 : Inport
  Atan2 : Trigonometry  Operator=atan2
  Cos : Trigonometry  Operator=cos
  Sin : Trigonometry
  Out1 : Outport
  wires:
  In1/1 -> Sin/1, Cos/1
  Cos/1 -> Atan2/2
  Atan2/1 -> Out1/1
  Sin/1 -> Atan2/1

== system Template_v5_0_0_2026a_Original/1 - Experiment Logic/Phase #3: Experiment/Sub-Phase #4/Desired Position BLACK/Calculate Circular Tracking ==
  Angular Frequency : Inport
  Phase : Inport  Port=2
  Constant1 : Constant  Value=xLength/2
  Constant2 : Constant  Value=yLength/2
  Cos : Trigonometry  Operator=cos
  Gain : Gain  Gain=0.85
  Gain1 : Gain  Gain=0.85
  Sin : Trigonometry
  Sum{,1..3} (4 alike) : Sum  Inputs=|++
  Target X : Outport
  Target Y : Outport  Port=2
  wires:
  Constant2/1 -> Sum2/2
  Constant1/1 -> Sum1/2
  Cos/1 -> Gain/1
  Gain1/1 -> Sum2/1
  Sin/1 -> Gain1/1
  Gain/1 -> Sum1/1
  Sum2/1 -> Target Y/1
  Sum1/1 -> Target X/1
  Angular Frequency/1 -> Sum3/1, Sum/1
  Sum/1 -> Cos/1
  Phase/1 -> Sum3/2, Sum/2
  Sum3/1 -> Sin/1

== system Template_v5_0_0_2026a_Original/1 - Experiment Logic/Phase #3: Experiment/Sub-Phase #4/Desired Position BLACK/Calculate Time since Phase #3 Start ==
  Constant2 : Constant  Value=Phase2_End  SampleTime=-1
  Subsystem : Subsystem
  Subtract3 : Sum  Inputs=+-
  Time : Outport  VectorParamsAs1DForOutWhenUnconnected=off
  wires:
  Subtract3/1 -> Time/1
  Constant2/1 -> Subtract3/2
  Subsystem/1(Time) -> Subtract3/1

== system Template_v5_0_0_2026a_Original/1 - Experiment Logic/Phase #3: Experiment/Sub-Phase #4/Desired Position BLACK/Wrap ==
  In1 : Inport
  Atan2 : Trigonometry  Operator=atan2
  Cos : Trigonometry  Operator=cos
  Sin : Trigonometry
  Out1 : Outport
  wires:
  In1/1 -> Sin/1, Cos/1
  Cos/1 -> Atan2/2
  Atan2/1 -> Out1/1
  Sin/1 -> Atan2/1

== system Template_v5_0_0_2026a_Original/1 - Experiment Logic/Phase #3: Experiment/Sub-Phase #4/Desired Position BLUE/Calculate Circular Tracking ==
  Angular Frequency : Inport
  Phase : Inport  Port=2
  Constant1 : Constant  Value=xLength/2
  Constant2 : Constant  Value=yLength/2
  Cos : Trigonometry  Operator=cos
  Gain : Gain  Gain=0.85
  Gain1 : Gain  Gain=0.85
  Sin : Trigonometry
  Sum{,1..3} (4 alike) : Sum  Inputs=|++
  Target X : Outport
  Target Y : Outport  Port=2
  wires:
  Constant2/1 -> Sum2/2
  Constant1/1 -> Sum1/2
  Cos/1 -> Gain/1
  Gain1/1 -> Sum2/1
  Sin/1 -> Gain1/1
  Gain/1 -> Sum1/1
  Sum2/1 -> Target Y/1
  Sum1/1 -> Target X/1
  Angular Frequency/1 -> Sum3/1, Sum/1
  Sum/1 -> Cos/1
  Phase/1 -> Sum3/2, Sum/2
  Sum3/1 -> Sin/1

== system Template_v5_0_0_2026a_Original/1 - Experiment Logic/Phase #3: Experiment/Sub-Phase #4/Desired Position BLUE/Calculate Time since Phase #3 Start ==
  Constant2 : Constant  Value=Phase2_End  SampleTime=-1
  Subsystem : Subsystem
  Subtract3 : Sum  Inputs=+-
  Time : Outport  VectorParamsAs1DForOutWhenUnconnected=off
  wires:
  Subtract3/1 -> Time/1
  Constant2/1 -> Subtract3/2
  Subsystem/1(Time) -> Subtract3/1

== system Template_v5_0_0_2026a_Original/1 - Experiment Logic/Phase #3: Experiment/Sub-Phase #4/Desired Position BLUE/Wrap ==
  In1 : Inport
  Atan2 : Trigonometry  Operator=atan2
  Cos : Trigonometry  Operator=cos
  Sin : Trigonometry
  Out1 : Outport
  wires:
  In1/1 -> Sin/1, Cos/1
  Cos/1 -> Atan2/2
  Atan2/1 -> Out1/1
  Sin/1 -> Atan2/1

== system Template_v5_0_0_2026a_Original/1 - Experiment Logic/Phase #3: Experiment/Sub-Phase #4/Desired Position RED/Calculate Circular Tracking ==
  Angular Frequency : Inport
  Phase : Inport  Port=2
  Constant1 : Constant  Value=xLength/2
  Constant2 : Constant  Value=yLength/2
  Cos : Trigonometry  Operator=cos
  Gain : Gain  Gain=0.85
  Gain1 : Gain  Gain=0.85
  Sin : Trigonometry
  Sum{,1..3} (4 alike) : Sum  Inputs=|++
  Target X : Outport
  Target Y : Outport  Port=2
  wires:
  Constant2/1 -> Sum2/2
  Constant1/1 -> Sum1/2
  Cos/1 -> Gain/1
  Gain1/1 -> Sum2/1
  Sin/1 -> Gain1/1
  Gain/1 -> Sum1/1
  Sum2/1 -> Target Y/1
  Sum1/1 -> Target X/1
  Angular Frequency/1 -> Sum3/1, Sum/1
  Sum/1 -> Cos/1
  Phase/1 -> Sum3/2, Sum/2
  Sum3/1 -> Sin/1

== system Template_v5_0_0_2026a_Original/1 - Experiment Logic/Phase #3: Experiment/Sub-Phase #4/Desired Position RED/Calculate Time since Phase #3 Start ==
  Constant2 : Constant  Value=Phase2_End  SampleTime=-1
  Subsystem : Subsystem
  Subtract3 : Sum  Inputs=+-
  Time : Outport  VectorParamsAs1DForOutWhenUnconnected=off
  wires:
  Subtract3/1 -> Time/1
  Constant2/1 -> Subtract3/2
  Subsystem/1(Time) -> Subtract3/1

== system Template_v5_0_0_2026a_Original/1 - Experiment Logic/Phase #3: Experiment/Sub-Phase #4/Desired Position RED/Wrap ==
  In1 : Inport
  Atan2 : Trigonometry  Operator=atan2
  Cos : Trigonometry  Operator=cos
  Sin : Trigonometry
  Out1 : Outport
  wires:
  In1/1 -> Sin/1, Cos/1
  Cos/1 -> Atan2/2
  Atan2/1 -> Out1/1
  Sin/1 -> Atan2/1

== system Template_v5_0_0_2026a_Original/PhaseSpace Camera Code/Use Hardware to Obtain States/Receive and Process Phasespace Data/Experiment Clock/Send Sync. Time ==
  Universal Time : Inport
  Change BLACK Behavior : Subsystem  TreatAsAtomicUnit=on
  Change BLUE Behavior : Subsystem  TreatAsAtomicUnit=on
  Change RED Behavior : Subsystem  TreatAsAtomicUnit=on
  Data Store Read : DataStoreRead  DataStoreName=WhoAmI  IndexOptions=Index vector (dialog)  Indices=1  OutputSizes=1
  Data Store Read2 : DataStoreRead  DataStoreName=isSim  IndexOptions=Index vector (dialog)  Indices=1  OutputSizes=1
  This IF block determines whether or not to run the BLACK sim/exp : If  NumInputs=2  IfExpression=u1 == 2 & u2 == 0  ShowElse=off
  This IF block determines whether or not to run the BLUE sim/exp : If  NumInputs=2  IfExpression=u1 == 3 & u2 == 0  ShowElse=off
  "This IF block determines whether or not to run the RED sim/exp " : If  NumInputs=2  IfExpression=u1 == 1 & u2 == 0  ShowElse=off
  wires:
  Data Store Read/1 -> This IF block determines whether or not to run the BLUE sim/exp/1, This IF block determines whether or not to run the BLACK sim/exp/1, "This IF block determines whether or not to run the RED sim/exp "/1
  This IF block determines whether or not to run the BLUE sim/exp/1 -> Change BLUE Behavior/Action
  "This IF block determines whether or not to run the RED sim/exp "/1 -> Change RED Behavior/Action
  Data Store Read2/1 -> This IF block determines whether or not to run the BLACK sim/exp/2, This IF block determines whether or not to run the BLUE sim/exp/2, "This IF block determines whether or not to run the RED sim/exp "/2
  This IF block determines whether or not to run the BLACK sim/exp/1 -> Change BLACK Behavior/Action
  Universal Time/1 -> Change BLACK Behavior/1(Universal Time), Change RED Behavior/1(Universal Time), Change BLUE Behavior/1(Universal Time)

== system Template_v5_0_0_2026a_Original/PhaseSpace Camera Code/Use Hardware to Obtain States/Store BLACK Data/Calculate True Time Step/Enabled Subsystem3 ==
  y2-y1 : Inport
  Enable : EnablePort
  dy(t)/dt : Outport
  wires:
  y2-y1/1 -> dy(t)/dt/1

== system Template_v5_0_0_2026a_Original/PhaseSpace Camera Code/Use Hardware to Obtain States/Store BLACK Data/Subsystem1/Enabled Subsystem ==
  y : Inport
  dt : Inport  Port=2
  Enable : EnablePort
  Constant2 : Constant  Value=0.1
  Delay : Delay  DelayLength=1
  MATLAB Function : MATLAB Function  TreatAsAtomicUnit=on
  dy/dt : Outport
  wires:
  Constant2/1 -> MATLAB Function/3(tau)
  dt/1 -> MATLAB Function/2(dt)
  Delay/1 -> MATLAB Function/4(ema_prev)
  MATLAB Function/2(ema) -> Delay/1
  y/1 -> MATLAB Function/1(y)
  MATLAB Function/1(dy) -> dy/dt/1

== system Template_v5_0_0_2026a_Original/PhaseSpace Camera Code/Use Hardware to Obtain States/Store BLACK Data/Subsystem2/Enabled Subsystem ==
  y : Inport
  dt : Inport  Port=2
  Enable : EnablePort
  Constant2 : Constant  Value=0.1
  Delay : Delay  DelayLength=1
  MATLAB Function : MATLAB Function  TreatAsAtomicUnit=on
  dy/dt : Outport
  wires:
  Constant2/1 -> MATLAB Function/3(tau)
  dt/1 -> MATLAB Function/2(dt)
  Delay/1 -> MATLAB Function/4(ema_prev)
  MATLAB Function/2(ema) -> Delay/1
  y/1 -> MATLAB Function/1(y)
  MATLAB Function/1(dy) -> dy/dt/1

== system Template_v5_0_0_2026a_Original/PhaseSpace Camera Code/Use Hardware to Obtain States/Store BLUE Data/Calculate True Time Step/Enabled Subsystem3 ==
  y2-y1 : Inport
  Enable : EnablePort
  dy(t)/dt : Outport
  wires:
  y2-y1/1 -> dy(t)/dt/1

== system Template_v5_0_0_2026a_Original/PhaseSpace Camera Code/Use Hardware to Obtain States/Store BLUE Data/Subsystem1/Enabled Subsystem ==
  y : Inport
  dt : Inport  Port=2
  Enable : EnablePort
  Constant2 : Constant  Value=0.1
  Delay : Delay  DelayLength=1
  MATLAB Function : MATLAB Function  TreatAsAtomicUnit=on
  dy/dt : Outport
  wires:
  Constant2/1 -> MATLAB Function/3(tau)
  dt/1 -> MATLAB Function/2(dt)
  Delay/1 -> MATLAB Function/4(ema_prev)
  MATLAB Function/2(ema) -> Delay/1
  y/1 -> MATLAB Function/1(y)
  MATLAB Function/1(dy) -> dy/dt/1

== system Template_v5_0_0_2026a_Original/PhaseSpace Camera Code/Use Hardware to Obtain States/Store BLUE Data/Subsystem2/Enabled Subsystem ==
  y : Inport
  dt : Inport  Port=2
  Enable : EnablePort
  Constant2 : Constant  Value=0.1
  Delay : Delay  DelayLength=1
  MATLAB Function : MATLAB Function  TreatAsAtomicUnit=on
  dy/dt : Outport
  wires:
  Constant2/1 -> MATLAB Function/3(tau)
  dt/1 -> MATLAB Function/2(dt)
  Delay/1 -> MATLAB Function/4(ema_prev)
  MATLAB Function/2(ema) -> Delay/1
  y/1 -> MATLAB Function/1(y)
  MATLAB Function/1(dy) -> dy/dt/1

== system Template_v5_0_0_2026a_Original/PhaseSpace Camera Code/Use Hardware to Obtain States/Store RED Data/Calculate True Time Step/Enabled Subsystem3 ==
  y2-y1 : Inport
  Enable : EnablePort
  dy(t)/dt : Outport
  wires:
  y2-y1/1 -> dy(t)/dt/1

== system Template_v5_0_0_2026a_Original/PhaseSpace Camera Code/Use Hardware to Obtain States/Store RED Data/Subsystem1/Enabled Subsystem ==
  y : Inport
  dt : Inport  Port=2
  Enable : EnablePort
  Constant2 : Constant  Value=0.1
  Delay : Delay  DelayLength=1
  MATLAB Function : MATLAB Function  TreatAsAtomicUnit=on
  dy/dt : Outport
  wires:
  Constant2/1 -> MATLAB Function/3(tau)
  dt/1 -> MATLAB Function/2(dt)
  Delay/1 -> MATLAB Function/4(ema_prev)
  MATLAB Function/2(ema) -> Delay/1
  y/1 -> MATLAB Function/1(y)
  MATLAB Function/1(dy) -> dy/dt/1

== system Template_v5_0_0_2026a_Original/PhaseSpace Camera Code/Use Hardware to Obtain States/Store RED Data/Subsystem2/Enabled Subsystem ==
  y : Inport
  dt : Inport  Port=2
  Enable : EnablePort
  Constant2 : Constant  Value=0.1
  Delay : Delay  DelayLength=1
  MATLAB Function : MATLAB Function  TreatAsAtomicUnit=on
  dy/dt : Outport
  wires:
  Constant2/1 -> MATLAB Function/3(tau)
  dt/1 -> MATLAB Function/2(dt)
  Delay/1 -> MATLAB Function/4(ema_prev)
  MATLAB Function/2(ema) -> Delay/1
  y/1 -> MATLAB Function/1(y)
  MATLAB Function/1(dy) -> dy/dt/1

== system Template_v5_0_0_2026a_Original/Simulate Plant Dynamics/BLACK Dynamics/Calculated & Store Measured States/Subsystem1/Enabled Subsystem ==
  y : Inport
  dt : Inport  Port=2
  Enable : EnablePort
  Constant2 : Constant  Value=0.1
  Delay : Delay  DelayLength=1
  MATLAB Function : MATLAB Function  TreatAsAtomicUnit=on
  dy/dt : Outport
  wires:
  Constant2/1 -> MATLAB Function/3(tau)
  dt/1 -> MATLAB Function/2(dt)
  Delay/1 -> MATLAB Function/4(ema_prev)
  MATLAB Function/2(ema) -> Delay/1
  y/1 -> MATLAB Function/1(y)
  MATLAB Function/1(dy) -> dy/dt/1

== system Template_v5_0_0_2026a_Original/Simulate Plant Dynamics/BLACK Dynamics/Calculated & Store Measured States/Subsystem2/Enabled Subsystem ==
  y : Inport
  dt : Inport  Port=2
  Enable : EnablePort
  Constant2 : Constant  Value=0.1
  Delay : Delay  DelayLength=1
  MATLAB Function : MATLAB Function  TreatAsAtomicUnit=on
  dy/dt : Outport
  wires:
  Constant2/1 -> MATLAB Function/3(tau)
  dt/1 -> MATLAB Function/2(dt)
  Delay/1 -> MATLAB Function/4(ema_prev)
  MATLAB Function/2(ema) -> Delay/1
  y/1 -> MATLAB Function/1(y)
  MATLAB Function/1(dy) -> dy/dt/1

== system Template_v5_0_0_2026a_Original/Simulate Plant Dynamics/BLACK Dynamics/Data @ Measurement Rate/Calculate True Time Step/Enabled Subsystem3 ==
  y2-y1 : Inport
  Enable : EnablePort
  dy(t)/dt : Outport
  wires:
  y2-y1/1 -> dy(t)/dt/1

== system Template_v5_0_0_2026a_Original/Simulate Plant Dynamics/BLUE Dynamics/Calculated & Store Measured States/Subsystem1/Enabled Subsystem ==
  y : Inport
  dt : Inport  Port=2
  Enable : EnablePort
  Constant2 : Constant  Value=0.1
  Delay : Delay  DelayLength=1
  MATLAB Function : MATLAB Function  TreatAsAtomicUnit=on
  dy/dt : Outport
  wires:
  Constant2/1 -> MATLAB Function/3(tau)
  dt/1 -> MATLAB Function/2(dt)
  Delay/1 -> MATLAB Function/4(ema_prev)
  MATLAB Function/2(ema) -> Delay/1
  y/1 -> MATLAB Function/1(y)
  MATLAB Function/1(dy) -> dy/dt/1

== system Template_v5_0_0_2026a_Original/Simulate Plant Dynamics/BLUE Dynamics/Calculated & Store Measured States/Subsystem2/Enabled Subsystem ==
  y : Inport
  dt : Inport  Port=2
  Enable : EnablePort
  Constant2 : Constant  Value=0.1
  Delay : Delay  DelayLength=1
  MATLAB Function : MATLAB Function  TreatAsAtomicUnit=on
  dy/dt : Outport
  wires:
  Constant2/1 -> MATLAB Function/3(tau)
  dt/1 -> MATLAB Function/2(dt)
  Delay/1 -> MATLAB Function/4(ema_prev)
  MATLAB Function/2(ema) -> Delay/1
  y/1 -> MATLAB Function/1(y)
  MATLAB Function/1(dy) -> dy/dt/1

== system Template_v5_0_0_2026a_Original/Simulate Plant Dynamics/BLUE Dynamics/Data @ Measurement Rate/Calculate True Time Step/Enabled Subsystem3 ==
  y2-y1 : Inport
  Enable : EnablePort
  dy(t)/dt : Outport
  wires:
  y2-y1/1 -> dy(t)/dt/1
